simulink model "PFC_TKDTCS"  (R2013a)
settings: Solver=ode45  StartTime=0.0  StopTime=0.35  RelTol=1e-3
libraries: powerlib x17, powerlib_meascontrol x1
settings Model: Creator=Mr. Nghia  LastModifiedBy=vuhoangphuong

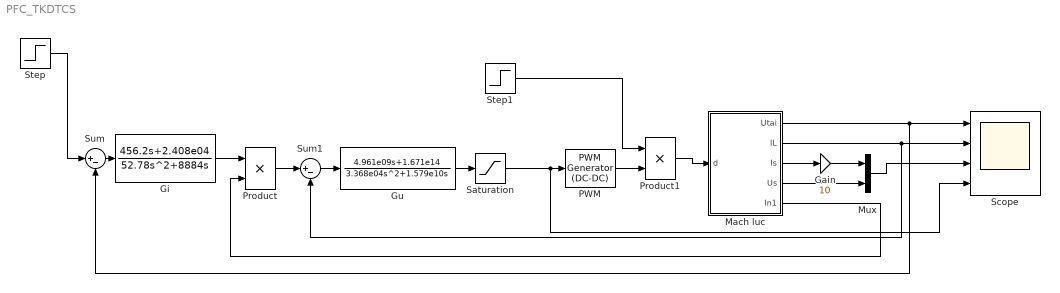
== system PFC_TKDTCS ==
  Gain : Gain  Gain=10
  Gi : TransferFcn  Numerator=[456.2 2.408e04]  Denominator=[52.78 8884 0]
  Gu : TransferFcn  Numerator=[4.961e09 1.671e14]  Denominator=[3.368e04 1.579e10 0]
  Mach luc : Subsystem
  Mux : Mux  Inputs=2
  PWM : powerlib_meascontrol/Pulse & Signal Generators/PWM Generator (DC-DC)  Fsw=100000  Ts=0
  Product : Product
  Product1 : Product
  Saturation : Saturate  UpperLimit=0.95  LowerLimit=0.01
  Scope : Scope  NumInputPorts=4
      settings: TimeRange=0.1  YMin=385~0~-350~0.1  YMax=425~10~350~1
  Step : Step  Time=0  After=400  SampleTime=0
  Step1 : Step  Time=0.05  SampleTime=0
  Sum : Sum  Inputs=|+-
  Sum1 : Sum  Inputs=|+-
  wires:
  Sum1/1 -> Gu/1
  Gu/1 -> Saturation/1
  Mach luc/1(Utai) -> Scope/1, Sum/2
  Mach luc/2("IL ") -> Scope/2, Sum1/2
  Mach luc/5(In1) -> Product/2
  Gi/1 -> Product/1
  Product/1 -> Sum1/1
  Sum/1 -> Gi/1
  PWM/1 -> Product1/2
  Product1/1 -> Mach luc/1("d ")
  Step1/1 -> Product1/1
  Mach luc/3("Is ") -> Gain/1
  Mach luc/4("Us ") -> Mux/2
  Mux/1 -> Scope/3
  Saturation/1 -> PWM/1, Scope/4
  Gain/1 -> Mux/1
  Step/1 -> Sum/1

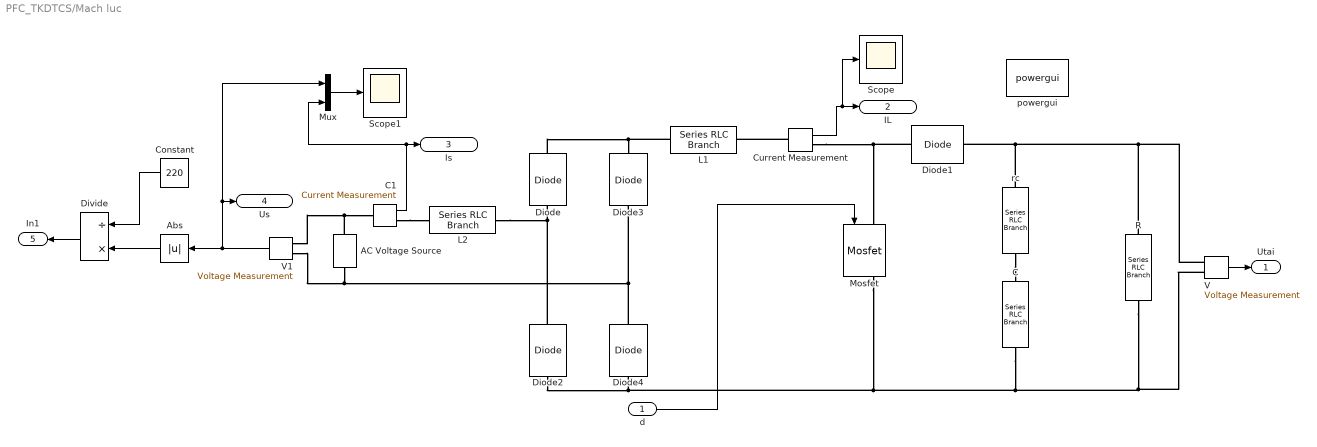
== system PFC_TKDTCS/Mach luc ==
  "d " : Inport
  AC Voltage Source : powerlib/Electrical Sources/AC Voltage Source  Amplitude=310  Phase=0  Frequency=50  SampleTime=0  Measurements=None
  Abs : Abs
  C : powerlib/Elements/Series RLC Branch  LConnTagsString=__new0  RConnTagsString=__new0  BranchType=C  Resistance=1  Inductance=1e-3  SetiL0=off  InitialCurrent=0  Capacitance=470e-6  Setx0=off  InitialVoltage=250  Measurements=None
  C1 : powerlib/Measurements/Current Measurement  PhasorSimulation=off  OutputType=Complex  PSBequivalent=0
  Constant : Constant  Value=220
  Current Measurement : powerlib/Measurements/Current Measurement  PhasorSimulation=off  OutputType=Complex  PSBequivalent=0
  Diode{,1..4} (5 alike) : powerlib/Power Electronics/Diode  Ron=0.001  Lon=0  Vf=0.8  IC=0  UseSnubber=off  Rs=500  Cs=250e-9  Measurements=off
  Divide : Product  Inputs=/*
  L1 : powerlib/Elements/Series RLC Branch  LConnTagsString=__new0  RConnTagsString=__new0  BranchType=L  Resistance=1  Inductance=1e-3  SetiL0=off  InitialCurrent=0  Capacitance=1e-6  Setx0=off  InitialVoltage=0  Measurements=None
  L2 : powerlib/Elements/Series RLC Branch  LConnTagsString=__new0  RConnTagsString=__new0  BranchType=L  Resistance=1  Inductance=1e-3  SetiL0=off  InitialCurrent=0  Capacitance=1e-6  Setx0=off  InitialVoltage=0  Measurements=None
  Mosfet : powerlib/Power Electronics/Mosfet  Ron=0.1  Lon=0  Rd=0.01  Vfd=0  IC=0  Rs=1e5  Cs=inf  Measurements=on
  Mux : Mux  Inputs=2
  R : powerlib/Elements/Series RLC Branch  LConnTagsString=__new0  RConnTagsString=__new0  BranchType=R  Resistance=160  Inductance=1e-3  SetiL0=off  InitialCurrent=0  Capacitance=1e-6  Setx0=off  InitialVoltage=0  Measurements=None
  Scope : Scope
      settings: TimeRange=0.1  YMin=0  YMax=16
  Scope1 : Scope
      settings: TimeRange=0.1  YMin=-225  YMax=225  SaveName=ScopeData2
  V : powerlib/Measurements/Voltage Measurement  PhasorSimulation=off  OutputType=Complex  PSBequivalent=0
  V1 : powerlib/Measurements/Voltage Measurement  PhasorSimulation=off  OutputType=Complex  PSBequivalent=0
  powergui : powerlib/powergui  Priority=1  SimulationMode=Continuous  SolverType=Tustin  SampleTime=50e-6  frequency=60  SPID=on  DisableSnubberDevices=off  DisableRonSwitches=off  DisableVfSwitches=off  SwTol=0  Interpol=off  DisplayEquations=off  frequencyindice=50  Pbase=100e6  ErrMax=1e-4  Iterations=50  UnitsV=kV  UnitsW=MW  FunctionMessages=off  echomessages=off  HookPort=off  EnableUseOfTLC=off  x0status=blocks  RestoreLinks=warning  ResistiveCurrentMeasurement=off  Frange=[0:2:500]  Ylog=off  Xlog=on  ShowGrid=off  save=off  variable=ZData  structure=ScopeData2  ZoomFFT=off  StartTime=0.3  cycles=1  DisplayStyle=1  fundamental=50  FreqAxis=on  MaxFrequency=10000  frequencyindicesteady=1  RmsSteady=1  display=off  Ts=0  methode=off
  rc : powerlib/Elements/Series RLC Branch  LConnTagsString=__new0  RConnTagsString=__new0  BranchType=R  Resistance=0.1  Inductance=1e-3  SetiL0=off  InitialCurrent=0  Capacitance=1e-6  Setx0=off  InitialVoltage=0  Measurements=None
  Utai : Outport
  "IL " : Outport  Port=2
  "Is " : Outport  Port=3
  "Us " : Outport  Port=4
  In1 : Outport  Port=5
  wires:
  "d "/1 -> Mosfet/1
  V/1 -> Utai/1
  Current Measurement/1 -> Scope/1, "IL "/1
  Constant/1 -> Divide/1
  Abs/1 -> Divide/2
  V1/1 -> Abs/1, Mux/1, "Us "/1
  Divide/1 -> In1/1
  C1/1 -> Mux/2, "Is "/1
  Mux/1 -> Scope1/1
  connections:
  Diode4/RConn1 -- V1/LConn2 -- AC Voltage Source/LConn1 -- Diode3/LConn1
  Diode2/RConn1 -- L2/RConn1 -- Diode/LConn1
  Diode/RConn1 -- L1/LConn1 -- Diode3/RConn1
  Diode2/LConn1 -- V/LConn2 -- R/RConn1 -- C/RConn1 -- Mosfet/RConn1 -- Diode4/LConn1
  Diode1/LConn1 -- Current Measurement/RConn1 -- Mosfet/LConn1
  R/LConn1 -- V/LConn1 -- rc/LConn1 -- Diode1/RConn1
  Current Measurement/LConn1 -- L1/RConn1
  AC Voltage Source/RConn1 -- V1/LConn1 -- C1/LConn1
  C1/RConn1 -- L2/LConn1
  rc/RConn1 -- C/LConn1
